simulink model "MascaraDigitalC4"  (R2024b)
settings: Solver=ode23tb  StartTime=0.0  StopTime=20  MaxStep=5e-3  RelTol=1e-3
InitFcn:
  | %% dados_cenarios.m  (revisado AP1)
  | % Sombra Digital - Ficha B4 (grupo gerador diesel, sistema isolado)
  | % Usina escalada a partir de Apui: 40 x UTE 550 + 10 transformadores.
  | % Rodar antes da simulacao ou chamar no InitFcn: run('dados_cenarios.m');
  | % Linhas marcadas com [REV] foram acrescentadas/alteradas na revisao.
  | 
  | %% 0) CENARIO (editar SOMENTE esta secao)
  | %   'C1' caso base (12 MW constantes, sem festividade)
  | %   'C2' curva de 24 h do CSV (perfil variavel; valores horarios por Load Flow, Secao 3.5)
  | %   'C3' festividade em regime (14 MW, banco ligado desde t = 0)
  | %   'C5' degrau da festividade: festa e banco fecham em t = t_evento (12 -> 14 MW)
  | %   'C6' perda de um bloco: maquina de 9 blocos + degrau de 1,435 MW em t = t_evento (equivale a perder 1 bloco)
  | cenario  = 'C1';
  | t_evento = 1;                           % s, instante do evento (C5 e C6)
  | 
  | % Chaves derivadas do cenario (nao editar)
  | fixar_base_lf = true;   evento_C5 = false;   evento_C6 = false;
  | N_sim = 10;             fest_estado_ini = 0; Pm0_est = 0.621859;        % Pm0_est: estimativa (usar o valor da mensagem do Load Flow)
  | switch cenario
  |     case 'C1'
  |     case 'C2', fixar_base_lf = false;
  |     case 'C3', fest_estado_ini = 1;  Pm0_est = 0.730088;
  |     case 'C5', evento_C5 = true;
  |     case 'C6', evento_C6 = true;  N_sim = 9;  Pm0_est = 0.691459;      % festa aberta; degrau resistivo em t_evento (Secao 14)
  |     otherwise, error('cenario invalido: use C1, C2, C3, C5 ou C6');
  | end
  | fprintf('=== Cenario %s | N_sim = %d | festa fechada em t0: %d ===\n', cenario, N_sim, fest_estado_ini);
  | 
  | %% 1) Solver e escala de tempo
  | Ts = 5e-5;                    % s. So e usado se o powergui voltar ao modo Discrete.
  | % seg_por_hora so e usado pelo perfil lido no From Workspace e pelos
  | % tempos do Breaker. Os valores horarios da AP2 sao obtidos por Load Flow
  | % hora a hora (Secao 3.5); os eventos C5 e C6 sao simulados por 20 s.
  | seg_por_hora = 1;             % 1 s simulado = 1 h (apenas para o perfil)
  | 
  | %% 2) Curva de carga 24 h (arquivo do professor)
  | T            = readtable('curva_carga_24h.csv');   % na pasta do modelo
  | horas        = double(T.hora(:));                  % 0..23 (em horas)
  | fator        = double(T.fator_carga(:));           % media = 0,804
  | temp_amb     = double(T.temp_ambiente_C(:));       % [REV] C, usada no derating
  | perfil_carga = [horas*seg_por_hora fator];         % Nx2 (tempo simulado, fator) -> From Workspace
  | assert(size(perfil_carga,1)==24 && size(perfil_carga,2)==2 && ...
  |        ~any(isnan(perfil_carga(:))), 'perfil_carga invalido: confira o CSV');
  | % Cenarios C1, C3, C5 e C6: carga constante no caso base (toda a curva em 1,0); C2 usa o perfil do CSV.
  | if fixar_base_lf, perfil_carga(:,2) = 1.0; end
  | 
  | %% 3) Geradores UTE 550 (regime Prime, ficha do fabricante [21])
  | S_unit   = 503e3;             % VA por gerador (Prime, ficha)
  | P_unit   = 0.8*S_unit;        % W, ~402,4 kW (FP nominal 0,8)
  | % [REV] Premissa: potencia aparente Prime da ficha x FP de placa; o consumo
  | % do ventilador eletrico nao e descontado (a ficha nao o informa).
  | N_ativos = 40;                % 10 blocos x 4 geradores  [ASSUNCAO de projeto]
  | Sn_usina = N_ativos*S_unit;   % 20,12 MVA
  | Pn_usina = N_ativos*P_unit;   % 16,10 MW
  | 
  | %% 4) Maquina sincrona equivalente (Synchronous Machine pu Standard)
  | Sn_maq = Sn_usina;            % VA (20,12 MVA com 10 blocos)
  | Vn_maq = 13.8e3;              % V. Maquina equivalente referida ao lado de 13,8 kV
  | % Nota: a usina real gera em 0,48 kV e eleva para 13,8 kV (trafos Dyn1).
  | % No modelo o gerador e referido ao lado de 13,8 kV (relacao 13,8/13,8 kV),
  | ... (+332 lines)
undefined symbols (not defined in the file or in its folder): D1, Delta, Pm0_gov
libraries: spsThreePhaseParallelRLCLoadLib x6, spsThreePhaseVIMeasurementLib x5, spsVoltageMeasurementLib x5, spsGroundLib x5, spsLoadFlowBusLib x4, spsThreePhaseDynamicLoadLib x3, spsThreePhaseSeriesRLCBranchLib x2, spsNeutralLib x2, spsRMSLib x2, spsThreePhaseBreakerLib x2, spsThreePhaseSeriesRLCLoadLib x1, spsExcitationSystemLib x1
(part 2 of 2)

== system MascaraDigitalC4/Info ==
